simulink model "dcsim_rt_hil"  (R2026a)
settings: Solver=FixedStepDiscrete  StopTime=inf  FixedStep=hil_dt
PreLoadFcn:
  | load(fullfile(fileparts(which('dcsim_rt_hil')), 'dcsim_rt_hil_data.mat'))
values from neighbouring files (symbols this model uses):
  pv = [800 132000 0.0242424242424 8e-05 0.0005 5e-06 0.005 0.008 640 0.0001 20 288.75 ... (36 elements, 36x1)]    [dcsim_rt_hil_data.mat]    (also in dcsim_rt_hil_demo.m = dcsim_rt_pv(shared, c); dcsim_rt_pv.m = [shared.V_ref; shared.P_rated; shared.R_droop; shared.tau_c;; hil_quickstart.m = evalin('base', 'pv'); rt_hil_check.m = dcsim_rt_pv(shared, c))
  qs_dt_min = 1.5e-6    (= 1.5e-06)    [run_rt_case.m]
  y0 = [797.942200076 84.8842468493 797.517778842 0 84.8842468493 797.263126102 67675.0799999 0.000903675421673 1320 50 0]    [dcsim_rt_hil_data.mat]    (also in dcsim_rt_hil_demo.m = dcsim_rt_hil_y0(pv_y0, P0, dt); dcsim_rt_hil_y0.m = y; dcsim_rt_init.m = [ic.v_c; ic.i_L; ic.v_C; ic.i_f; ic.i_Lin; ic.v_Cin; ic.P_cm; run_hil_handover.m = dcsim_rt_hil_y0(pv_y0, 0.5 * shared.P_rated, dt))
undefined symbols (not defined in the file or in its folder): ao_fs_V, ao_pu_1, ao_pu_2, ao_pu_3, ao_pu_4, brk_delay, conv_smooth, fault_arc_m, fault_arc_ramp, fault_Lf, fault_Lf48, fault_mode, fault_Rf, fault_Rf48, fault_trigger, fault_type, fault_Varc, hil_dt, rearm_cmd, run_enable, step_dP, step_ramp, sync_width, uvlo_tol, wl_dP1, wl_dP2, wl_duty1, wl_duty2, wl_jit1, wl_jit2, wl_on, wl_P0, wl_ramp1, wl_ramp2, wl_seed, wl_T1, wl_T2
Description:
  | dcsim_rt_hil build 2026-10-16 (MODEL.md 0.4.4 + breaker element rev 2, HIL wrapper rev 2: review fixes #1-#13)
settings Model: Creator=USER  LastModifiedBy=USER

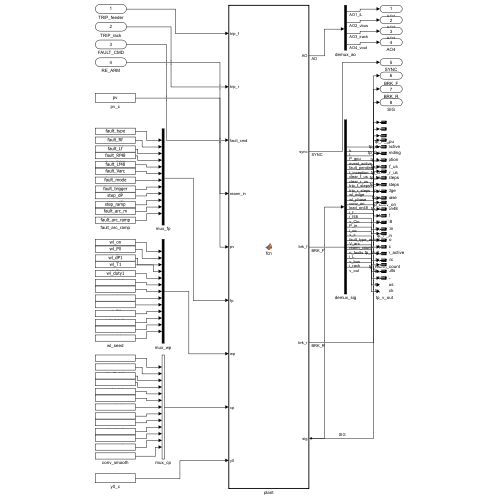
[thumbnail: Simulink's stored preview of the top-level diagram]
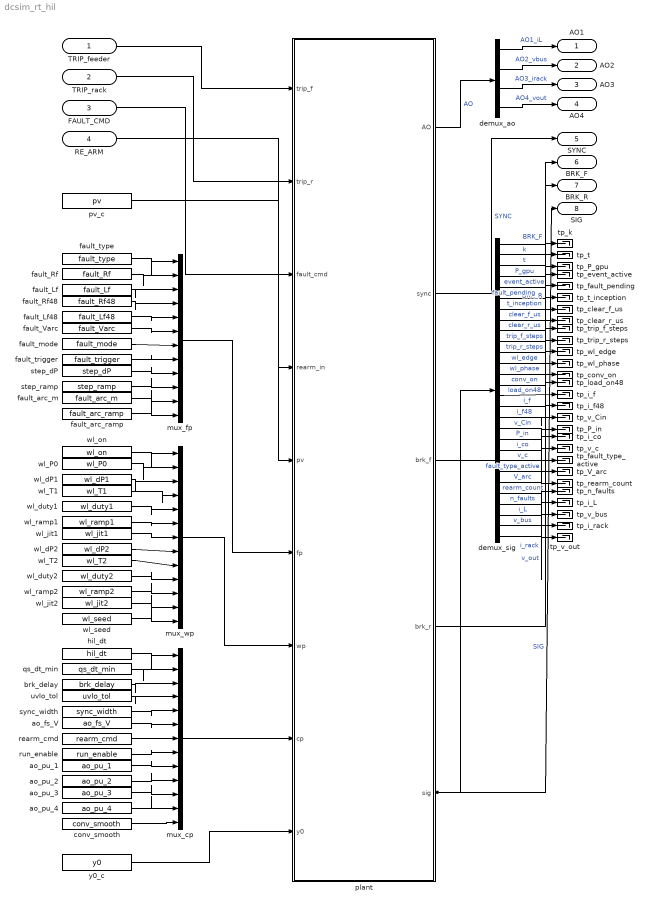
== system dcsim_rt_hil ==
  TRIP_feeder : Inport  SampleTime=hil_dt
  TRIP_rack : Inport  Port=2  SampleTime=hil_dt
  FAULT_CMD : Inport  Port=3  SampleTime=hil_dt
  RE_ARM : Inport  Port=4  SampleTime=hil_dt
  ao_fs_V : Constant  Value=ao_fs_V  SampleTime=hil_dt
  ao_pu_1 : Constant  Value=ao_pu_1  SampleTime=hil_dt
  ao_pu_2 : Constant  Value=ao_pu_2  SampleTime=hil_dt
  ao_pu_3 : Constant  Value=ao_pu_3  SampleTime=hil_dt
  ao_pu_4 : Constant  Value=ao_pu_4  SampleTime=hil_dt
  brk_delay : Constant  Value=brk_delay  SampleTime=hil_dt
  conv_smooth : Constant  Value=conv_smooth  SampleTime=hil_dt
  demux_ao : Demux
  demux_sig : Demux  Outputs=28
  fault_Lf : Constant  Value=fault_Lf  SampleTime=hil_dt
  fault_Lf48 : Constant  Value=fault_Lf48  SampleTime=hil_dt
  fault_Rf : Constant  Value=fault_Rf  SampleTime=hil_dt
  fault_Rf48 : Constant  Value=fault_Rf48  SampleTime=hil_dt
  fault_Varc : Constant  Value=fault_Varc  SampleTime=hil_dt
  fault_arc_m : Constant  Value=fault_arc_m  SampleTime=hil_dt
  fault_arc_ramp : Constant  Value=fault_arc_ramp  SampleTime=hil_dt
  fault_mode : Constant  Value=fault_mode  SampleTime=hil_dt
  fault_trigger : Constant  Value=fault_trigger  SampleTime=hil_dt
  fault_type : Constant  Value=fault_type  SampleTime=hil_dt
  hil_dt : Constant  Value=hil_dt  SampleTime=hil_dt
  mux_cp : Mux  Inputs=13
  mux_fp : Mux  Inputs=12
  mux_wp : Mux  Inputs=13
  plant : MATLAB Function  TreatAsAtomicUnit=on
  pv_c : Constant  Value=pv  SampleTime=hil_dt
  qs_dt_min : Constant  Value=qs_dt_min  SampleTime=hil_dt
  rearm_cmd : Constant  Value=rearm_cmd  SampleTime=hil_dt
  run_enable : Constant  Value=run_enable  SampleTime=hil_dt
  step_dP : Constant  Value=step_dP  SampleTime=hil_dt
  step_ramp : Constant  Value=step_ramp  SampleTime=hil_dt
  sync_width : Constant  Value=sync_width  SampleTime=hil_dt
  tp_P_gpu : Terminator
  tp_P_in : Terminator
  tp_V_arc : Terminator
  tp_clear_f_us : Terminator
  tp_clear_r_us : Terminator
  tp_conv_on : Terminator
  tp_event_active : Terminator
  tp_fault_pending : Terminator
  tp_fault_type_active : Terminator
  tp_i_L : Terminator
  tp_i_co : Terminator
  tp_i_f : Terminator
  tp_i_f48 : Terminator
  tp_i_rack : Terminator
  tp_k : Terminator
  tp_load_on48 : Terminator
  tp_n_faults : Terminator
  tp_rearm_count : Terminator
  tp_t : Terminator
  tp_t_inception : Terminator
  tp_trip_f_steps : Terminator
  tp_trip_r_steps : Terminator
  tp_v_Cin : Terminator
  tp_v_bus : Terminator
  tp_v_c : Terminator
  tp_v_out : Terminator
  tp_wl_edge : Terminator
  tp_wl_phase : Terminator
  uvlo_tol : Constant  Value=uvlo_tol  SampleTime=hil_dt
  wl_P0 : Constant  Value=wl_P0  SampleTime=hil_dt
  wl_T1 : Constant  Value=wl_T1  SampleTime=hil_dt
  wl_T2 : Constant  Value=wl_T2  SampleTime=hil_dt
  wl_dP1 : Constant  Value=wl_dP1  SampleTime=hil_dt
  wl_dP2 : Constant  Value=wl_dP2  SampleTime=hil_dt
  wl_duty1 : Constant  Value=wl_duty1  SampleTime=hil_dt
  wl_duty2 : Constant  Value=wl_duty2  SampleTime=hil_dt
  wl_jit1 : Constant  Value=wl_jit1  SampleTime=hil_dt
  wl_jit2 : Constant  Value=wl_jit2  SampleTime=hil_dt
  wl_on : Constant  Value=wl_on  SampleTime=hil_dt
  wl_ramp1 : Constant  Value=wl_ramp1  SampleTime=hil_dt
  wl_ramp2 : Constant  Value=wl_ramp2  SampleTime=hil_dt
  wl_seed : Constant  Value=wl_seed  SampleTime=hil_dt
  y0_c : Constant  Value=y0  SampleTime=hil_dt
  AO1 : Outport
  AO2 : Outport  Port=2
  AO3 : Outport  Port=3
  AO4 : Outport  Port=4
  SYNC : Outport  Port=5
  BRK_F : Outport  Port=6
  BRK_R : Outport  Port=7
  SIG : Outport  Port=8
  wires:
  fault_type/1 -> mux_fp/1
  fault_Rf/1 -> mux_fp/2
  fault_Lf/1 -> mux_fp/3
  fault_Rf48/1 -> mux_fp/4
  fault_Lf48/1 -> mux_fp/5
  fault_Varc/1 -> mux_fp/6
  fault_mode/1 -> mux_fp/7
  fault_trigger/1 -> mux_fp/8
  step_dP/1 -> mux_fp/9
  step_ramp/1 -> mux_fp/10
  fault_arc_m/1 -> mux_fp/11
  fault_arc_ramp/1 -> mux_fp/12
  wl_on/1 -> mux_wp/1
  wl_P0/1 -> mux_wp/2
  wl_dP1/1 -> mux_wp/3
  wl_T1/1 -> mux_wp/4
  wl_duty1/1 -> mux_wp/5
  wl_ramp1/1 -> mux_wp/6
  wl_jit1/1 -> mux_wp/7
  wl_dP2/1 -> mux_wp/8
  wl_T2/1 -> mux_wp/9
  wl_duty2/1 -> mux_wp/10
  wl_ramp2/1 -> mux_wp/11
  wl_jit2/1 -> mux_wp/12
  wl_seed/1 -> mux_wp/13
  hil_dt/1 -> mux_cp/1
  qs_dt_min/1 -> mux_cp/2
  brk_delay/1 -> mux_cp/3
  uvlo_tol/1 -> mux_cp/4
  sync_width/1 -> mux_cp/5
  ao_fs_V/1 -> mux_cp/6
  rearm_cmd/1 -> mux_cp/7
  run_enable/1 -> mux_cp/8
  ao_pu_1/1 -> mux_cp/9
  ao_pu_2/1 -> mux_cp/10
  ao_pu_3/1 -> mux_cp/11
  ao_pu_4/1 -> mux_cp/12
  conv_smooth/1 -> mux_cp/13
  TRIP_feeder/1 -> plant/1(trip_f)
  TRIP_rack/1 -> plant/2(trip_r)
  FAULT_CMD/1 -> plant/3(fault_cmd)
  RE_ARM/1 -> plant/4(rearm_in)
  pv_c/1 -> plant/5(pv)
  mux_fp/1 -> plant/6(fp)
  mux_wp/1 -> plant/7(wp)
  mux_cp/1 -> plant/8(cp)
  y0_c/1 -> plant/9(y0)
  plant/1(AO) -> demux_ao/1  "AO"
  demux_ao/1 -> AO1/1  "AO1_iL"
  demux_ao/2 -> AO2/1  "AO2_vbus"
  demux_ao/3 -> AO3/1  "AO3_irack"
  demux_ao/4 -> AO4/1  "AO4_vout"
  plant/2(sync) -> SYNC/1  "SYNC"
  plant/3(brk_f) -> BRK_F/1  "BRK_F"
  plant/4(brk_r) -> BRK_R/1  "BRK_R"
  plant/5(sig) -> SIG/1, demux_sig/1  "SIG"
  demux_sig/1 -> tp_k/1  "k"
  demux_sig/2 -> tp_t/1  "t"
  demux_sig/3 -> tp_P_gpu/1  "P_gpu"
  demux_sig/4 -> tp_event_active/1  "event_active"
  demux_sig/5 -> tp_fault_pending/1  "fault_pending"
  demux_sig/6 -> tp_t_inception/1  "t_inception"
  demux_sig/7 -> tp_clear_f_us/1  "clear_f_us"
  demux_sig/8 -> tp_clear_r_us/1  "clear_r_us"
  demux_sig/9 -> tp_trip_f_steps/1  "trip_f_steps"
  demux_sig/10 -> tp_trip_r_steps/1  "trip_r_steps"
  demux_sig/11 -> tp_wl_edge/1  "wl_edge"
  demux_sig/12 -> tp_wl_phase/1  "wl_phase"
  demux_sig/13 -> tp_conv_on/1  "conv_on"
  demux_sig/14 -> tp_load_on48/1  "load_on48"
  demux_sig/15 -> tp_i_f/1  "i_f"
  demux_sig/16 -> tp_i_f48/1  "i_f48"
  demux_sig/17 -> tp_v_Cin/1  "v_Cin"
  demux_sig/18 -> tp_P_in/1  "P_in"
  demux_sig/19 -> tp_i_co/1  "i_co"
  demux_sig/20 -> tp_v_c/1  "v_c"
  demux_sig/21 -> tp_fault_type_active/1  "fault_type_active"
  demux_sig/22 -> tp_V_arc/1  "V_arc"
  demux_sig/23 -> tp_rearm_count/1  "rearm_count"
  demux_sig/24 -> tp_n_faults/1  "n_faults"
  demux_sig/25 -> tp_i_L/1  "i_L"
  demux_sig/26 -> tp_v_bus/1  "v_bus"
  demux_sig/27 -> tp_i_rack/1  "i_rack"
  demux_sig/28 -> tp_v_out/1  "v_out"

== matlab function dcsim_rt_hil/plant ==
  data: trip_f input; AO output; trip_r input; fault_cmd input; rearm_in input; pv input; fp input; wp input; cp input; y0 input; sync output; brk_f output; brk_r output; sig output
function [AO, sync, brk_f, brk_r, sig] = plant(trip_f, trip_r, fault_cmd, rearm_in, pv, fp, wp, cp, y0)
%#codegen
[AO, sync, brk_f, brk_r, sig] = dcsim_rt_hil_plant(trip_f, trip_r, fault_cmd, rearm_in, pv, fp, wp, cp, y0);
end
